simulink model "Model_RE_Load_RECTIFIER_battery10x2820x29_night"  (R2024b)
settings: Solver=ode23t  StartTime=0.0  StopTime=1  MaxStep=1e-3  RelTol=1e-3
undefined symbols (not defined in the file): Ion, Lithium
libraries: spsSeriesRLCBranchLib x6, spsIGBTDiodeLib x4, spsMultimeterLib x4, spsMeanLib x4, spsDiodeLib x4, spsCurrentMeasurementLib x2, spsVoltageMeasurementLib x2, spsACVoltageSourceLib x1, spsPWMGeneratorDCDCLib x1, spsBatteryLib x1, spsMutualInductanceLib x1, spsPowerLib x1
settings Model: Creator=Arjun TM  LastModifiedBy=hello
settings SolverCC: AlgebraicLoopSolver=TrustRegion
settings DataIOCC: ReturnWorkspaceOutputs=off
settings DebuggingCC: UnconnectedInputMsg=warning  UnconnectedOutputMsg=warning  UnconnectedLineMsg=warning
settings ModelReferenceCC: EnableRefExpFcnMdlSchedulingChecks=on
settings RTWCC: GPUComputeCapability=3.5  DLArmComputeVersion=19.05

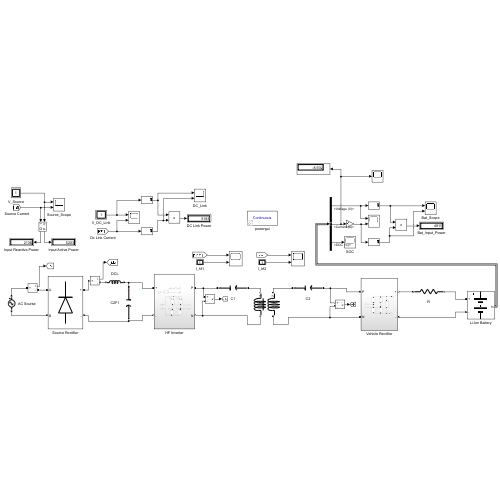
[thumbnail: Simulink's stored preview of the top-level diagram]
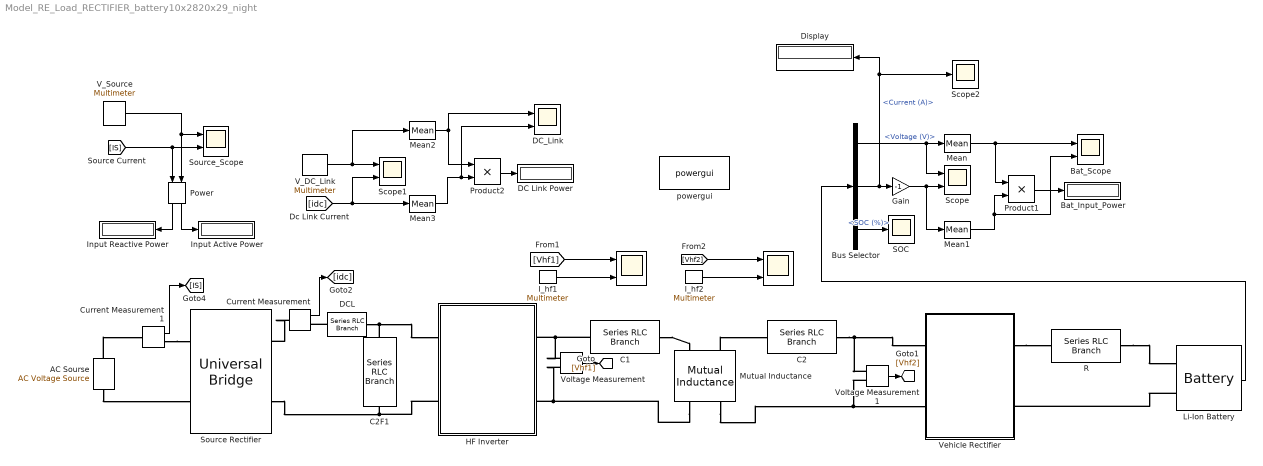
== system Model_RE_Load_RECTIFIER_battery10x2820x29_night ==
  " " : Scope  NumInputPorts=2
  "   " : Scope  NumInputPorts=2
  AC Sourse : spsACVoltageSourceLib/AC Voltage Source  Amplitude=325  Phase=0  Frequency=50  SampleTime=0  Measurements=Voltage  BusType=swing  Pref=10e3  Qref=0  Qmin=-inf  Qmax=+inf
  Bat_Input_Power : Display
  Bat_Scope : Scope  NumInputPorts=2
  Bus Selector : BusSelector  OutputSignals=Voltage (V),Current (A),SOC (%)
  C1 : spsSeriesRLCBranchLib/Series RLC Branch  LConnTagsString=__new0  RConnTagsString=__new0  BranchType=C  Resistance=1e-6  Inductance=1e-3  SetiL0=off  InitialCurrent=0  Capacitance=105.74e-9  Setx0=off  InitialVoltage=0  Measurements=Branch current
  C2 : spsSeriesRLCBranchLib/Series RLC Branch  LConnTagsString=__new0  RConnTagsString=__new0  BranchType=C  Resistance=1e-6  Inductance=1e-3  SetiL0=off  InitialCurrent=0  Capacitance=109.69e-9  Setx0=off  InitialVoltage=0  Measurements=Branch current
  C2F1 : spsSeriesRLCBranchLib/Series RLC Branch  LConnTagsString=__new0  RConnTagsString=__new0  BranchType=C  Resistance=1e-6  Inductance=1e-3  SetiL0=off  InitialCurrent=0  Capacitance=300e-6  Setx0=off  InitialVoltage=0  Measurements=None
  Current Measurement : spsCurrentMeasurementLib/Current Measurement  PhasorSimulation=off  OutputType=Complex  PSBequivalent=0
  Current Measurement1 : spsCurrentMeasurementLib/Current Measurement  PhasorSimulation=off  OutputType=Complex  PSBequivalent=0
  DC Link Power : Display
  DCL : spsSeriesRLCBranchLib/Series RLC Branch  LConnTagsString=__new0  RConnTagsString=__new0  BranchType=L  Resistance=0.1  Inductance=10e-3  SetiL0=off  InitialCurrent=0  Capacitance=1e-6  Setx0=off  InitialVoltage=0  Measurements=Branch current
  DC_Link : Scope  NumInputPorts=2
  Display : Display
  Gain : Gain  Gain=-1
  HF Inverter : Subsystem
  I_hf1 : spsMultimeterLib/Multimeter  L=15  sel=9  yselected={}  Gain=1  OutputType=Complex  PlotAtSimulationStop=off  PhasorSimulation=off
  I_hf2 : spsMultimeterLib/Multimeter  L=15  sel=10  yselected={}  Gain=1  OutputType=Complex  PlotAtSimulationStop=off  PhasorSimulation=off
  Input Active Power : Display
  Input Reactive Power : Display
  Li-Ion Battery : spsBatteryLib/Battery  BatType=Lithium-Ion  NomV=350  NomQ=115  SOC=90  Batt_Tr=10  PresetModel=on  MaxQ=115  MinV=262.5  FullV=407.3955  Dis_rate=50  R=0.030435  Normal_OP=104  expZone="[378.135          5.65]"
      settings: LibrarySourceBlock=electricdrivelib/Extra Sources/Battery
  Mean{,1..3} (4 alike) : spsMeanLib/Mean  Freq=50  Vinit=0  Ts=0
  Mutual Inductance : spsMutualInductanceLib/Mutual Inductance  LConnTagsString=a|b  RConnTagsString=A|B  TypeOfMutual=Two or three windings with equal mutual terms  NumberOfWindings=3  SelfImpedance1=[1e-3 266.16e-6]  SelfImpedance2=[1e-3 256.79e-6]  ThreeWindings=off  SelfImpedance3=[ 1.1 1.1e-03]  MutualImpedance=[0 85.46e-6]  InductanceMatrix="[1.0 0.9  0.9 ;  0.9 1.0  0.9;  0.9 0.9 1.0 ] * 1e-3"  ResistanceMatrix="[1.0 0.9  0.9 ;  0.9 1.0  0.9;  0.9 0.9 1.0 ]"  Measurements=None
      settings: LibrarySourceBlock=sps_lib/Passives/Mutual Inductance
  Power : spsPowerLib/Power  Freq=50  Vinit=[1, 0]  Iinit=[1, 0]  Ts=0
  Product1 : Product
  Product2 : Product
  R : spsSeriesRLCBranchLib/Series RLC Branch  LConnTagsString=__new0  RConnTagsString=__new0  BranchType=R  Resistance=0.01  Inductance=1e-3  SetiL0=off  InitialCurrent=0  Capacitance=1e-6  Setx0=off  InitialVoltage=0  Measurements=None
  SOC : Scope
  Scope : Scope  NumInputPorts=2
  Scope1 : Scope  NumInputPorts=2
  Scope2 : Scope
  Source Rectifier : spsUniversalBridgeLib/Universal Bridge  Arms=2  SnubberResistance=1e5  SnubberCapacitance=inf  Device=Diodes  Ron=1e-3  Lon=0  ForwardVoltages="[  0  0  ]"  ForwardVoltage=0  GTOparameters=[ 10e-6 , 20e-6 ]  IGBTparameters=[ 1e-6 , 2e-6 ]  Measurements=All voltages and currents  Measurements_2=None  converterType=Rectifier
  Source_Scope : Scope  NumInputPorts=2
  V_DC_Link : spsMultimeterLib/Multimeter  L=15  sel=7  yselected={}  Gain=1  OutputType=Complex  PlotAtSimulationStop=off  PhasorSimulation=off
  V_Source : spsMultimeterLib/Multimeter  L=15  sel=8  yselected={}  Gain=1  OutputType=Complex  PlotAtSimulationStop=off  PhasorSimulation=off
  Vehicle Rectifier : Subsystem
  Voltage Measurement : spsVoltageMeasurementLib/Voltage Measurement  PhasorSimulation=off  OutputType=Complex  PSBequivalent=0
  Voltage Measurement1 : spsVoltageMeasurementLib/Voltage Measurement  PhasorSimulation=off  OutputType=Complex  PSBequivalent=0
  powergui : spspowerguiLib/powergui  Priority=1  SimulationMode=Continuous  SampleTime=50e-6  frequency=60  Iterations=50  frequencyindice=0  Pbase=100e6  ErrMax=1e-4  UnitsV=kV  UnitsW=MW  buscounter=0  FunctionMessages=off  echomessages=off  EnableUseOfTLC=off  CurrentSourceSwitches=off  DisableSnubberDevices=off  DisableRonSwitches=off  DisableVfSwitches=off  DisplayEquations=off  AutomaticDiscreteSolvers=off  SolverType=Tustin/Backward Euler (TBE)  Interpol=off  ExternalGateDelay=off  methode=off  Ts=100  x0status=blocks  SPID=on  SwTol=0  HookPort=off  NonlinearTolerance=1e-4  nMaxIteration=100  ContinueOnMaxIteration=off  RestoreLinks=warning  ResistiveCurrentMeasurement=off  Frange=[0:2:500]  Ylog=off  Xlog=on  ShowGrid=off  save=off  variable=ZData  structure=source  ZoomFFT=off  StartTime=0.1  cycles=5  DisplayStyle=2  fundamental=50  FreqAxis=on  MaxFrequency=1000  frequencyindicesteady=1  RmsSteady=1  display=off
  wires:
  Product1/1 -> Bat_Input_Power/1
  Mean/1 -> Bat_Scope/1, Product1/1
  Mean1/1 -> Bat_Scope/2, Product1/2
  Current Measurement/1 -> [idc]
  V_Source/1 -> Source_Scope/1, Power/1
  Power/1 -> Input Active Power/1
  [IS] -> Power/2, Source_Scope/2
  Current Measurement1/1 -> [IS]
  Power/2 -> Input Reactive Power/1
  Mean3/1 -> DC_Link/2, Product2/2
  Mean2/1 -> DC_Link/1, Product2/1
  Product2/1 -> DC Link Power/1
  [idc] -> Mean3/1, Scope1/2
  V_DC_Link/1 -> Mean2/1, Scope1/1
  Voltage Measurement/1 -> [Vhf1]
  Voltage Measurement1/1 -> [Vhf2]
  [Vhf1] -> " "/1
  I_hf1/1 -> " "/2
  I_hf2/1 -> "   "/2
  [Vhf2] -> "   "/1
  Li-Ion Battery/1 -> Bus Selector/1
  Bus Selector/1 -> Scope/1, Mean/1  "<Voltage (V)>"
  Bus Selector/2 -> Scope2/1, Display/1, Gain/1  "<Current (A)>"
  Gain/1 -> Mean1/1, Scope/2
  Bus Selector/3 -> SOC/1  "<SOC (%)>"
  connections:
  C1/RConn1 -- Mutual Inductance/LConn1
  Mutual Inductance/LConn2 -- C2/LConn1
  AC Sourse/LConn1 -- Source Rectifier/LConn2
  Current Measurement/LConn1 -- Source Rectifier/RConn1
  AC Sourse/RConn1 -- Current Measurement1/LConn1
  Current Measurement1/RConn1 -- Source Rectifier/LConn1
  Source Rectifier/RConn2 -- HF Inverter/LConn2 -- C2F1/RConn1
  C2F1/LConn1 -- DCL/LConn1 -- HF Inverter/LConn1
  C1/LConn1 -- Voltage Measurement/LConn1 -- HF Inverter/RConn1
  Mutual Inductance/RConn1 -- Voltage Measurement/LConn2 -- HF Inverter/RConn2
  C2/RConn1 -- Voltage Measurement1/LConn1 -- Vehicle Rectifier/LConn1
  Mutual Inductance/RConn2 -- Voltage Measurement1/LConn2 -- Vehicle Rectifier/LConn2
  DCL/RConn1 -- Current Measurement/RConn1
  Li-Ion Battery/LConn2 -- Vehicle Rectifier/RConn2
  Vehicle Rectifier/RConn1 -- R/LConn1
  R/RConn1 -- Li-Ion Battery/LConn1

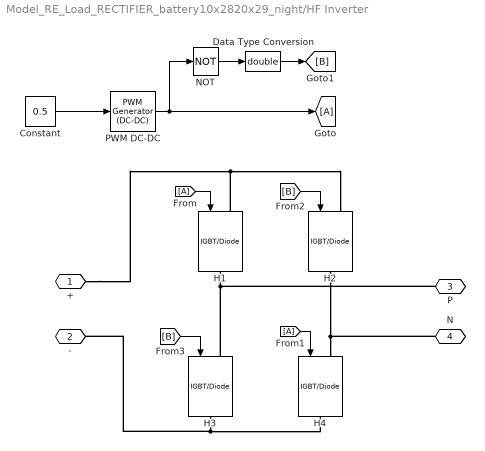
== system Model_RE_Load_RECTIFIER_battery10x2820x29_night/HF Inverter ==
  Constant : Constant  Value=0.5
  Data Type Conversion : DataTypeConversion  OutDataTypeStr=double  SaturateOnIntegerOverflow=off  RndMeth=Floor
  From : From
  From1 : From
  Goto : Goto
  H{1..4} (4 alike) : spsIGBTDiodeLib/IGBT//Diode  Ron=1e-3  Rs=1e5  Cs=inf  Measurements=off
  "NOT " : Logic  Operator=NOT  IconShape=distinctive  AllPortsSameDT=off  OutDataTypeStr=boolean
  PWM DC-DC : spsPWMGeneratorDCDCLib/PWM Generator (DC-DC)  Fsw=30000  Ts=0
  + : PMIOPort  Side=Left
  - : PMIOPort  Port=2  Side=Left
  P : PMIOPort  Port=3  Side=Right
  N : PMIOPort  Port=4  Side=Right
  wires:
  [B] -> H2/1
  [B] -> H3/1
  From1/1 -> H4/1
  From/1 -> H1/1
  "NOT "/1 -> Data Type Conversion/1
  Constant/1 -> PWM DC-DC/1
  Data Type Conversion/1 -> [B]
  PWM DC-DC/1 -> "NOT "/1, Goto/1
  connections:
  H1/LConn1 -- H2/LConn1 -- +/RConn1
  H2/RConn1 -- N/RConn1 -- H4/LConn1
  H3/RConn1 -- -/RConn1 -- H4/RConn1
  H3/LConn1 -- P/RConn1 -- H1/RConn1

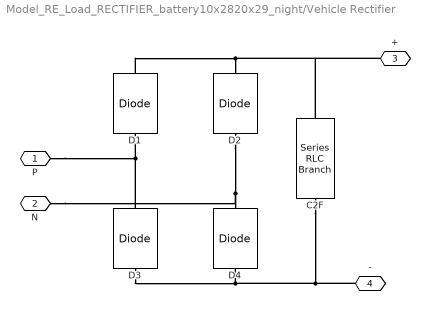
== system Model_RE_Load_RECTIFIER_battery10x2820x29_night/Vehicle Rectifier ==
  C2F : spsSeriesRLCBranchLib/Series RLC Branch  LConnTagsString=__new0  RConnTagsString=__new0  BranchType=C  Resistance=1e-6  Inductance=1e-3  SetiL0=off  InitialCurrent=0  Capacitance=300e-6  Setx0=off  InitialVoltage=0  Measurements=Branch voltage
  D{1..4} (4 alike) : spsDiodeLib/Diode  Ron=0.001  Lon=0  Vf=0.8  IC=0  UseSnubber=0  Rs=500  Cs=250e-9  Measurements=off
  P : PMIOPort  Side=Left
  N : PMIOPort  Port=2  Side=Left
  + : PMIOPort  Port=3  Side=Right
  - : PMIOPort  Port=4  Side=Right
  connections:
  D1/RConn1 -- +/RConn1 -- C2F/LConn1 -- D2/RConn1
  D3/RConn1 -- P/RConn1 -- D1/LConn1
  C2F/RConn1 -- -/RConn1 -- D3/LConn1 -- D4/LConn1
  D2/LConn1 -- N/RConn1 -- D4/RConn1
